simulink library "lib_LargeBuildingModel"  (R2026a)
settings: Solver=VariableStepAuto
libraries: WallSelector_lib x380, ExternalWall_lib x188, RoomWithAirVolume x140, fl_lib x139, RoomLevelControl_lib x1
(part 4 of 12)

== system lib_LargeBuildingModel/LargeBuildingModelLib/ConnectLevel3and4 ==
  note: Floor_A13R1(LivingRoom_A)
  note: Floor_A13R2(Bedroom_A)
  note: Floor_A13R3(Kitchen_A)
  note: Floor_A13R4(Bathroom_A)
  note: Floor_A13R5(FireExit_A)
  note: Floor_A13R6(Lobby1_A)
  note: Floor_A13R7(Lobby2_A)
  note: Floor_A14R1(LivingRoom_B)
  note: Floor_A14R2(Bedroom_B)
  note: Floor_A14R3(Kitchen_B)
  note: Floor_A14R4(Bathroom_B)
  note: Floor_A14R5(FireExit_B)
  note: Floor_A14R6(Lobby1_B)
  note: Floor_A14R7(Lobby2_B)
  note: Floor_A15R1(LivingRoom_C)
  note: Floor_A15R2(Bedroom_C)
  note: Floor_A15R3(Kitchen_C)
  note: Floor_A15R4(Bathroom_C)
  note: Floor_A15R5(FireExit_C)
  note: Floor_A15R6(Lobby1_C)
  note: Floor_A15R7(Lobby2_C)
  note: Floor_A16R1(LivingRoom_D)
  note: Floor_A16R2(Bedroom_D)
  note: Floor_A16R3(Kitchen_D)
  note: Floor_A16R4(Bathroom_D)
  note: Floor_A16R5(FireExit_D)
  note: Floor_A16R6(Lobby1_D)
  note: Floor_A16R7(Lobby2_D)
  ArrayBottom : SimscapeArrayConnection  Domain=foundation.thermal.thermal  ConcatenateDimension=1  NumScalarElements=28
  ArrayTop : SimscapeArrayConnection  Domain=foundation.thermal.thermal  ConcatenateDimension=1  NumScalarElements=28
  Floor_A13R1(LivingRoom_A)Blk : WallSelector_lib/Wall Selector  optWall=wallModelOption.wallOnly  wallLength=2.4384 % Parameterized on : 13-Jun-2026 10:47:16 m  wallHeight=4.572 % Parameterized on : 13-Jun-2026 10:47:16 m  wallThickness=0.03 % Parameterized on : 13-Jun-2026 10:47:16 m  wallMaterialDen=1400 % Parameterized on : 13-Jun-2026 10:47:30 kg/m^3  wallMaterialCp=1000 % Parameterized on : 13-Jun-2026 10:47:30 J/(K*kg)  wallAbsorptivity=0.5  wallThermalK=0.7 % Parameterized on : 13-Jun-2026 10:47:30 W/(K*m)  winLength=1 m  winHeight=0.5 m  winThickness=0.007 m  winMaterialDen=2500 kg/m^3  winMaterialCp=787 J/(K*kg)  winAbsorptivity=0.35  winThermalK=1 W/(K*m)  winTransmissivity=0.45  ventLength=0.1 m  ventHeight=0.1 m  extToWallHTC=30 % Parameterized on : 13-Jun-2026 10:47:30 W/(K*m^2)  intToRoomHTC=30 % Parameterized on : 13-Jun-2026 10:47:30 W/(K*m^2)  iniT=300 % Parameterized on : 13-Jun-2026 10:47:30 K
  Floor_A13R2(Bedroom_A)Blk : WallSelector_lib/Wall Selector  optWall=wallModelOption.wallOnly  wallLength=4.2672 % Parameterized on : 13-Jun-2026 10:47:16 m  wallHeight=4.572 % Parameterized on : 13-Jun-2026 10:47:16 m  wallThickness=0.03 % Parameterized on : 13-Jun-2026 10:47:16 m  wallMaterialDen=1400 % Parameterized on : 13-Jun-2026 10:47:30 kg/m^3  wallMaterialCp=1000 % Parameterized on : 13-Jun-2026 10:47:30 J/(K*kg)  wallAbsorptivity=0.5  wallThermalK=0.7 % Parameterized on : 13-Jun-2026 10:47:30 W/(K*m)  winLength=1 m  winHeight=0.5 m  winThickness=0.007 m  winMaterialDen=2500 kg/m^3  winMaterialCp=787 J/(K*kg)  winAbsorptivity=0.35  winThermalK=1 W/(K*m)  winTransmissivity=0.45  ventLength=0.1 m  ventHeight=0.1 m  extToWallHTC=30 % Parameterized on : 13-Jun-2026 10:47:30 W/(K*m^2)  intToRoomHTC=30 % Parameterized on : 13-Jun-2026 10:47:30 W/(K*m^2)  iniT=300 % Parameterized on : 13-Jun-2026 10:47:30 K
  Floor_A13R3(Kitchen_A)Blk : WallSelector_lib/Wall Selector  optWall=wallModelOption.wallOnly  wallLength=2.7432 % Parameterized on : 13-Jun-2026 10:47:16 m  wallHeight=3.9624 % Parameterized on : 13-Jun-2026 10:47:16 m  wallThickness=0.03 % Parameterized on : 13-Jun-2026 10:47:16 m  wallMaterialDen=1400 % Parameterized on : 13-Jun-2026 10:47:30 kg/m^3  wallMaterialCp=1000 % Parameterized on : 13-Jun-2026 10:47:30 J/(K*kg)  wallAbsorptivity=0.5  wallThermalK=0.7 % Parameterized on : 13-Jun-2026 10:47:30 W/(K*m)  winLength=1 m  winHeight=0.5 m  winThickness=0.007 m  winMaterialDen=2500 kg/m^3  winMaterialCp=787 J/(K*kg)  winAbsorptivity=0.35  winThermalK=1 W/(K*m)  winTransmissivity=0.45  ventLength=0.1 m  ventHeight=0.1 m  extToWallHTC=30 % Parameterized on : 13-Jun-2026 10:47:30 W/(K*m^2)  intToRoomHTC=30 % Parameterized on : 13-Jun-2026 10:47:30 W/(K*m^2)  iniT=300 % Parameterized on : 13-Jun-2026 10:47:30 K
  Floor_A13R4(Bathroom_A)Blk : WallSelector_lib/Wall Selector  optWall=wallModelOption.wallOnly  wallLength=2.4384 % Parameterized on : 13-Jun-2026 10:47:16 m  wallHeight=3.6576 % Parameterized on : 13-Jun-2026 10:47:16 m  wallThickness=0.03 % Parameterized on : 13-Jun-2026 10:47:16 m  wallMaterialDen=1400 % Parameterized on : 13-Jun-2026 10:47:30 kg/m^3  wallMaterialCp=1000 % Parameterized on : 13-Jun-2026 10:47:30 J/(K*kg)  wallAbsorptivity=0.5  wallThermalK=0.7 % Parameterized on : 13-Jun-2026 10:47:30 W/(K*m)  winLength=1 m  winHeight=0.5 m  winThickness=0.007 m  winMaterialDen=2500 kg/m^3  winMaterialCp=787 J/(K*kg)  winAbsorptivity=0.35  winThermalK=1 W/(K*m)  winTransmissivity=0.45  ventLength=0.1 m  ventHeight=0.1 m  extToWallHTC=30 % Parameterized on : 13-Jun-2026 10:47:30 W/(K*m^2)  intToRoomHTC=30 % Parameterized on : 13-Jun-2026 10:47:30 W/(K*m^2)  iniT=300 % Parameterized on : 13-Jun-2026 10:47:30 K
  Floor_A13R5(FireExit_A)Blk : WallSelector_lib/Wall Selector  optWall=wallModelOption.wallOnly  wallLength=1.8288 % Parameterized on : 13-Jun-2026 10:47:16 m  wallHeight=2.1336 % Parameterized on : 13-Jun-2026 10:47:16 m  wallThickness=0.03 % Parameterized on : 13-Jun-2026 10:47:16 m  wallMaterialDen=1400 % Parameterized on : 13-Jun-2026 10:47:30 kg/m^3  wallMaterialCp=1000 % Parameterized on : 13-Jun-2026 10:47:30 J/(K*kg)  wallAbsorptivity=0.5  wallThermalK=0.7 % Parameterized on : 13-Jun-2026 10:47:30 W/(K*m)  winLength=1 m  winHeight=0.5 m  winThickness=0.007 m  winMaterialDen=2500 kg/m^3  winMaterialCp=787 J/(K*kg)  winAbsorptivity=0.35  winThermalK=1 W/(K*m)  winTransmissivity=0.45  ventLength=0.1 m  ventHeight=0.1 m  extToWallHTC=30 % Parameterized on : 13-Jun-2026 10:47:30 W/(K*m^2)  intToRoomHTC=30 % Parameterized on : 13-Jun-2026 10:47:30 W/(K*m^2)  iniT=300 % Parameterized on : 13-Jun-2026 10:47:30 K
  Floor_A13R6(Lobby1_A)Blk : WallSelector_lib/Wall Selector  optWall=wallModelOption.wallOnly  wallLength=2.4384 % Parameterized on : 13-Jun-2026 10:47:16 m  wallHeight=2.4384 % Parameterized on : 13-Jun-2026 10:47:16 m  wallThickness=0.03 % Parameterized on : 13-Jun-2026 10:47:16 m  wallMaterialDen=1400 % Parameterized on : 13-Jun-2026 10:47:30 kg/m^3  wallMaterialCp=1000 % Parameterized on : 13-Jun-2026 10:47:30 J/(K*kg)  wallAbsorptivity=0.5  wallThermalK=0.7 % Parameterized on : 13-Jun-2026 10:47:30 W/(K*m)  winLength=1 m  winHeight=0.5 m  winThickness=0.007 m  winMaterialDen=2500 kg/m^3  winMaterialCp=787 J/(K*kg)  winAbsorptivity=0.35  winThermalK=1 W/(K*m)  winTransmissivity=0.45  ventLength=0.1 m  ventHeight=0.1 m  extToWallHTC=30 % Parameterized on : 13-Jun-2026 10:47:30 W/(K*m^2)  intToRoomHTC=30 % Parameterized on : 13-Jun-2026 10:47:30 W/(K*m^2)  iniT=300 % Parameterized on : 13-Jun-2026 10:47:30 K
  Floor_A13R7(Lobby2_A)Blk : WallSelector_lib/Wall Selector  optWall=wallModelOption.wallOnly  wallLength=2.4384 % Parameterized on : 13-Jun-2026 10:47:16 m  wallHeight=1.524 % Parameterized on : 13-Jun-2026 10:47:16 m  wallThickness=0.03 % Parameterized on : 13-Jun-2026 10:47:16 m  wallMaterialDen=1400 % Parameterized on : 13-Jun-2026 10:47:30 kg/m^3  wallMaterialCp=1000 % Parameterized on : 13-Jun-2026 10:47:30 J/(K*kg)  wallAbsorptivity=0.5  wallThermalK=0.7 % Parameterized on : 13-Jun-2026 10:47:30 W/(K*m)  winLength=1 m  winHeight=0.5 m  winThickness=0.007 m  winMaterialDen=2500 kg/m^3  winMaterialCp=787 J/(K*kg)  winAbsorptivity=0.35  winThermalK=1 W/(K*m)  winTransmissivity=0.45  ventLength=0.1 m  ventHeight=0.1 m  extToWallHTC=30 % Parameterized on : 13-Jun-2026 10:47:30 W/(K*m^2)  intToRoomHTC=30 % Parameterized on : 13-Jun-2026 10:47:30 W/(K*m^2)  iniT=300 % Parameterized on : 13-Jun-2026 10:47:30 K
  Floor_A14R1(LivingRoom_B)Blk : WallSelector_lib/Wall Selector  optWall=wallModelOption.wallOnly  wallLength=2.4384 % Parameterized on : 13-Jun-2026 10:47:16 m  wallHeight=4.572 % Parameterized on : 13-Jun-2026 10:47:16 m  wallThickness=0.03 % Parameterized on : 13-Jun-2026 10:47:16 m  wallMaterialDen=1400 % Parameterized on : 13-Jun-2026 10:47:30 kg/m^3  wallMaterialCp=1000 % Parameterized on : 13-Jun-2026 10:47:30 J/(K*kg)  wallAbsorptivity=0.5  wallThermalK=0.7 % Parameterized on : 13-Jun-2026 10:47:30 W/(K*m)  winLength=1 m  winHeight=0.5 m  winThickness=0.007 m  winMaterialDen=2500 kg/m^3  winMaterialCp=787 J/(K*kg)  winAbsorptivity=0.35  winThermalK=1 W/(K*m)  winTransmissivity=0.45  ventLength=0.1 m  ventHeight=0.1 m  extToWallHTC=30 % Parameterized on : 13-Jun-2026 10:47:30 W/(K*m^2)  intToRoomHTC=30 % Parameterized on : 13-Jun-2026 10:47:30 W/(K*m^2)  iniT=300 % Parameterized on : 13-Jun-2026 10:47:30 K
  Floor_A14R2(Bedroom_B)Blk : WallSelector_lib/Wall Selector  optWall=wallModelOption.wallOnly  wallLength=4.2672 % Parameterized on : 13-Jun-2026 10:47:16 m  wallHeight=4.572 % Parameterized on : 13-Jun-2026 10:47:16 m  wallThickness=0.03 % Parameterized on : 13-Jun-2026 10:47:16 m  wallMaterialDen=1400 % Parameterized on : 13-Jun-2026 10:47:30 kg/m^3  wallMaterialCp=1000 % Parameterized on : 13-Jun-2026 10:47:30 J/(K*kg)  wallAbsorptivity=0.5  wallThermalK=0.7 % Parameterized on : 13-Jun-2026 10:47:30 W/(K*m)  winLength=1 m  winHeight=0.5 m  winThickness=0.007 m  winMaterialDen=2500 kg/m^3  winMaterialCp=787 J/(K*kg)  winAbsorptivity=0.35  winThermalK=1 W/(K*m)  winTransmissivity=0.45  ventLength=0.1 m  ventHeight=0.1 m  extToWallHTC=30 % Parameterized on : 13-Jun-2026 10:47:30 W/(K*m^2)  intToRoomHTC=30 % Parameterized on : 13-Jun-2026 10:47:30 W/(K*m^2)  iniT=300 % Parameterized on : 13-Jun-2026 10:47:30 K
  Floor_A14R3(Kitchen_B)Blk : WallSelector_lib/Wall Selector  optWall=wallModelOption.wallOnly  wallLength=2.7432 % Parameterized on : 13-Jun-2026 10:47:16 m  wallHeight=3.9624 % Parameterized on : 13-Jun-2026 10:47:16 m  wallThickness=0.03 % Parameterized on : 13-Jun-2026 10:47:16 m  wallMaterialDen=1400 % Parameterized on : 13-Jun-2026 10:47:30 kg/m^3  wallMaterialCp=1000 % Parameterized on : 13-Jun-2026 10:47:30 J/(K*kg)  wallAbsorptivity=0.5  wallThermalK=0.7 % Parameterized on : 13-Jun-2026 10:47:30 W/(K*m)  winLength=1 m  winHeight=0.5 m  winThickness=0.007 m  winMaterialDen=2500 kg/m^3  winMaterialCp=787 J/(K*kg)  winAbsorptivity=0.35  winThermalK=1 W/(K*m)  winTransmissivity=0.45  ventLength=0.1 m  ventHeight=0.1 m  extToWallHTC=30 % Parameterized on : 13-Jun-2026 10:47:30 W/(K*m^2)  intToRoomHTC=30 % Parameterized on : 13-Jun-2026 10:47:30 W/(K*m^2)  iniT=300 % Parameterized on : 13-Jun-2026 10:47:30 K
  Floor_A14R4(Bathroom_B)Blk : WallSelector_lib/Wall Selector  optWall=wallModelOption.wallOnly  wallLength=2.4384 % Parameterized on : 13-Jun-2026 10:47:16 m  wallHeight=3.6576 % Parameterized on : 13-Jun-2026 10:47:16 m  wallThickness=0.03 % Parameterized on : 13-Jun-2026 10:47:16 m  wallMaterialDen=1400 % Parameterized on : 13-Jun-2026 10:47:30 kg/m^3  wallMaterialCp=1000 % Parameterized on : 13-Jun-2026 10:47:30 J/(K*kg)  wallAbsorptivity=0.5  wallThermalK=0.7 % Parameterized on : 13-Jun-2026 10:47:30 W/(K*m)  winLength=1 m  winHeight=0.5 m  winThickness=0.007 m  winMaterialDen=2500 kg/m^3  winMaterialCp=787 J/(K*kg)  winAbsorptivity=0.35  winThermalK=1 W/(K*m)  winTransmissivity=0.45  ventLength=0.1 m  ventHeight=0.1 m  extToWallHTC=30 % Parameterized on : 13-Jun-2026 10:47:30 W/(K*m^2)  intToRoomHTC=30 % Parameterized on : 13-Jun-2026 10:47:30 W/(K*m^2)  iniT=300 % Parameterized on : 13-Jun-2026 10:47:30 K
  Floor_A14R5(FireExit_B)Blk : WallSelector_lib/Wall Selector  optWall=wallModelOption.wallOnly  wallLength=1.8288 % Parameterized on : 13-Jun-2026 10:47:16 m  wallHeight=2.1336 % Parameterized on : 13-Jun-2026 10:47:16 m  wallThickness=0.03 % Parameterized on : 13-Jun-2026 10:47:16 m  wallMaterialDen=1400 % Parameterized on : 13-Jun-2026 10:47:30 kg/m^3  wallMaterialCp=1000 % Parameterized on : 13-Jun-2026 10:47:30 J/(K*kg)  wallAbsorptivity=0.5  wallThermalK=0.7 % Parameterized on : 13-Jun-2026 10:47:30 W/(K*m)  winLength=1 m  winHeight=0.5 m  winThickness=0.007 m  winMaterialDen=2500 kg/m^3  winMaterialCp=787 J/(K*kg)  winAbsorptivity=0.35  winThermalK=1 W/(K*m)  winTransmissivity=0.45  ventLength=0.1 m  ventHeight=0.1 m  extToWallHTC=30 % Parameterized on : 13-Jun-2026 10:47:30 W/(K*m^2)  intToRoomHTC=30 % Parameterized on : 13-Jun-2026 10:47:30 W/(K*m^2)  iniT=300 % Parameterized on : 13-Jun-2026 10:47:30 K
  Floor_A14R6(Lobby1_B)Blk : WallSelector_lib/Wall Selector  optWall=wallModelOption.wallOnly  wallLength=2.4384 % Parameterized on : 13-Jun-2026 10:47:16 m  wallHeight=2.4384 % Parameterized on : 13-Jun-2026 10:47:16 m  wallThickness=0.03 % Parameterized on : 13-Jun-2026 10:47:16 m  wallMaterialDen=1400 % Parameterized on : 13-Jun-2026 10:47:30 kg/m^3  wallMaterialCp=1000 % Parameterized on : 13-Jun-2026 10:47:30 J/(K*kg)  wallAbsorptivity=0.5  wallThermalK=0.7 % Parameterized on : 13-Jun-2026 10:47:30 W/(K*m)  winLength=1 m  winHeight=0.5 m  winThickness=0.007 m  winMaterialDen=2500 kg/m^3  winMaterialCp=787 J/(K*kg)  winAbsorptivity=0.35  winThermalK=1 W/(K*m)  winTransmissivity=0.45  ventLength=0.1 m  ventHeight=0.1 m  extToWallHTC=30 % Parameterized on : 13-Jun-2026 10:47:30 W/(K*m^2)  intToRoomHTC=30 % Parameterized on : 13-Jun-2026 10:47:30 W/(K*m^2)  iniT=300 % Parameterized on : 13-Jun-2026 10:47:30 K
  Floor_A14R7(Lobby2_B)Blk : WallSelector_lib/Wall Selector  optWall=wallModelOption.wallOnly  wallLength=2.4384 % Parameterized on : 13-Jun-2026 10:47:16 m  wallHeight=1.524 % Parameterized on : 13-Jun-2026 10:47:16 m  wallThickness=0.03 % Parameterized on : 13-Jun-2026 10:47:16 m  wallMaterialDen=1400 % Parameterized on : 13-Jun-2026 10:47:30 kg/m^3  wallMaterialCp=1000 % Parameterized on : 13-Jun-2026 10:47:30 J/(K*kg)  wallAbsorptivity=0.5  wallThermalK=0.7 % Parameterized on : 13-Jun-2026 10:47:30 W/(K*m)  winLength=1 m  winHeight=0.5 m  winThickness=0.007 m  winMaterialDen=2500 kg/m^3  winMaterialCp=787 J/(K*kg)  winAbsorptivity=0.35  winThermalK=1 W/(K*m)  winTransmissivity=0.45  ventLength=0.1 m  ventHeight=0.1 m  extToWallHTC=30 % Parameterized on : 13-Jun-2026 10:47:30 W/(K*m^2)  intToRoomHTC=30 % Parameterized on : 13-Jun-2026 10:47:30 W/(K*m^2)  iniT=300 % Parameterized on : 13-Jun-2026 10:47:30 K
  Floor_A15R1(LivingRoom_C)Blk : WallSelector_lib/Wall Selector  optWall=wallModelOption.wallOnly  wallLength=2.4384 % Parameterized on : 13-Jun-2026 10:47:16 m  wallHeight=4.572 % Parameterized on : 13-Jun-2026 10:47:16 m  wallThickness=0.03 % Parameterized on : 13-Jun-2026 10:47:16 m  wallMaterialDen=1400 % Parameterized on : 13-Jun-2026 10:47:30 kg/m^3  wallMaterialCp=1000 % Parameterized on : 13-Jun-2026 10:47:30 J/(K*kg)  wallAbsorptivity=0.5  wallThermalK=0.7 % Parameterized on : 13-Jun-2026 10:47:30 W/(K*m)  winLength=1 m  winHeight=0.5 m  winThickness=0.007 m  winMaterialDen=2500 kg/m^3  winMaterialCp=787 J/(K*kg)  winAbsorptivity=0.35  winThermalK=1 W/(K*m)  winTransmissivity=0.45  ventLength=0.1 m  ventHeight=0.1 m  extToWallHTC=30 % Parameterized on : 13-Jun-2026 10:47:30 W/(K*m^2)  intToRoomHTC=30 % Parameterized on : 13-Jun-2026 10:47:30 W/(K*m^2)  iniT=300 % Parameterized on : 13-Jun-2026 10:47:30 K
  Floor_A15R2(Bedroom_C)Blk : WallSelector_lib/Wall Selector  optWall=wallModelOption.wallOnly  wallLength=4.2672 % Parameterized on : 13-Jun-2026 10:47:16 m  wallHeight=4.572 % Parameterized on : 13-Jun-2026 10:47:16 m  wallThickness=0.03 % Parameterized on : 13-Jun-2026 10:47:16 m  wallMaterialDen=1400 % Parameterized on : 13-Jun-2026 10:47:30 kg/m^3  wallMaterialCp=1000 % Parameterized on : 13-Jun-2026 10:47:30 J/(K*kg)  wallAbsorptivity=0.5  wallThermalK=0.7 % Parameterized on : 13-Jun-2026 10:47:30 W/(K*m)  winLength=1 m  winHeight=0.5 m  winThickness=0.007 m  winMaterialDen=2500 kg/m^3  winMaterialCp=787 J/(K*kg)  winAbsorptivity=0.35  winThermalK=1 W/(K*m)  winTransmissivity=0.45  ventLength=0.1 m  ventHeight=0.1 m  extToWallHTC=30 % Parameterized on : 13-Jun-2026 10:47:30 W/(K*m^2)  intToRoomHTC=30 % Parameterized on : 13-Jun-2026 10:47:30 W/(K*m^2)  iniT=300 % Parameterized on : 13-Jun-2026 10:47:30 K
  Floor_A15R3(Kitchen_C)Blk : WallSelector_lib/Wall Selector  optWall=wallModelOption.wallOnly  wallLength=2.7432 % Parameterized on : 13-Jun-2026 10:47:16 m  wallHeight=3.9624 % Parameterized on : 13-Jun-2026 10:47:16 m  wallThickness=0.03 % Parameterized on : 13-Jun-2026 10:47:16 m  wallMaterialDen=1400 % Parameterized on : 13-Jun-2026 10:47:30 kg/m^3  wallMaterialCp=1000 % Parameterized on : 13-Jun-2026 10:47:30 J/(K*kg)  wallAbsorptivity=0.5  wallThermalK=0.7 % Parameterized on : 13-Jun-2026 10:47:30 W/(K*m)  winLength=1 m  winHeight=0.5 m  winThickness=0.007 m  winMaterialDen=2500 kg/m^3  winMaterialCp=787 J/(K*kg)  winAbsorptivity=0.35  winThermalK=1 W/(K*m)  winTransmissivity=0.45  ventLength=0.1 m  ventHeight=0.1 m  extToWallHTC=30 % Parameterized on : 13-Jun-2026 10:47:30 W/(K*m^2)  intToRoomHTC=30 % Parameterized on : 13-Jun-2026 10:47:30 W/(K*m^2)  iniT=300 % Parameterized on : 13-Jun-2026 10:47:30 K
  Floor_A15R4(Bathroom_C)Blk : WallSelector_lib/Wall Selector  optWall=wallModelOption.wallOnly  wallLength=2.4384 % Parameterized on : 13-Jun-2026 10:47:16 m  wallHeight=3.6576 % Parameterized on : 13-Jun-2026 10:47:16 m  wallThickness=0.03 % Parameterized on : 13-Jun-2026 10:47:16 m  wallMaterialDen=1400 % Parameterized on : 13-Jun-2026 10:47:30 kg/m^3  wallMaterialCp=1000 % Parameterized on : 13-Jun-2026 10:47:30 J/(K*kg)  wallAbsorptivity=0.5  wallThermalK=0.7 % Parameterized on : 13-Jun-2026 10:47:30 W/(K*m)  winLength=1 m  winHeight=0.5 m  winThickness=0.007 m  winMaterialDen=2500 kg/m^3  winMaterialCp=787 J/(K*kg)  winAbsorptivity=0.35  winThermalK=1 W/(K*m)  winTransmissivity=0.45  ventLength=0.1 m  ventHeight=0.1 m  extToWallHTC=30 % Parameterized on : 13-Jun-2026 10:47:30 W/(K*m^2)  intToRoomHTC=30 % Parameterized on : 13-Jun-2026 10:47:30 W/(K*m^2)  iniT=300 % Parameterized on : 13-Jun-2026 10:47:30 K
  Floor_A15R5(FireExit_C)Blk : WallSelector_lib/Wall Selector  optWall=wallModelOption.wallOnly  wallLength=1.8288 % Parameterized on : 13-Jun-2026 10:47:16 m  wallHeight=2.1336 % Parameterized on : 13-Jun-2026 10:47:16 m  wallThickness=0.03 % Parameterized on : 13-Jun-2026 10:47:16 m  wallMaterialDen=1400 % Parameterized on : 13-Jun-2026 10:47:30 kg/m^3  wallMaterialCp=1000 % Parameterized on : 13-Jun-2026 10:47:30 J/(K*kg)  wallAbsorptivity=0.5  wallThermalK=0.7 % Parameterized on : 13-Jun-2026 10:47:30 W/(K*m)  winLength=1 m  winHeight=0.5 m  winThickness=0.007 m  winMaterialDen=2500 kg/m^3  winMaterialCp=787 J/(K*kg)  winAbsorptivity=0.35  winThermalK=1 W/(K*m)  winTransmissivity=0.45  ventLength=0.1 m  ventHeight=0.1 m  extToWallHTC=30 % Parameterized on : 13-Jun-2026 10:47:30 W/(K*m^2)  intToRoomHTC=30 % Parameterized on : 13-Jun-2026 10:47:30 W/(K*m^2)  iniT=300 % Parameterized on : 13-Jun-2026 10:47:30 K
  Floor_A15R6(Lobby1_C)Blk : WallSelector_lib/Wall Selector  optWall=wallModelOption.wallOnly  wallLength=2.4384 % Parameterized on : 13-Jun-2026 10:47:16 m  wallHeight=2.4384 % Parameterized on : 13-Jun-2026 10:47:16 m  wallThickness=0.03 % Parameterized on : 13-Jun-2026 10:47:16 m  wallMaterialDen=1400 % Parameterized on : 13-Jun-2026 10:47:30 kg/m^3  wallMaterialCp=1000 % Parameterized on : 13-Jun-2026 10:47:30 J/(K*kg)  wallAbsorptivity=0.5  wallThermalK=0.7 % Parameterized on : 13-Jun-2026 10:47:30 W/(K*m)  winLength=1 m  winHeight=0.5 m  winThickness=0.007 m  winMaterialDen=2500 kg/m^3  winMaterialCp=787 J/(K*kg)  winAbsorptivity=0.35  winThermalK=1 W/(K*m)  winTransmissivity=0.45  ventLength=0.1 m  ventHeight=0.1 m  extToWallHTC=30 % Parameterized on : 13-Jun-2026 10:47:30 W/(K*m^2)  intToRoomHTC=30 % Parameterized on : 13-Jun-2026 10:47:30 W/(K*m^2)  iniT=300 % Parameterized on : 13-Jun-2026 10:47:30 K
  Floor_A15R7(Lobby2_C)Blk : WallSelector_lib/Wall Selector  optWall=wallModelOption.wallOnly  wallLength=2.4384 % Parameterized on : 13-Jun-2026 10:47:16 m  wallHeight=1.524 % Parameterized on : 13-Jun-2026 10:47:16 m  wallThickness=0.03 % Parameterized on : 13-Jun-2026 10:47:16 m  wallMaterialDen=1400 % Parameterized on : 13-Jun-2026 10:47:30 kg/m^3  wallMaterialCp=1000 % Parameterized on : 13-Jun-2026 10:47:30 J/(K*kg)  wallAbsorptivity=0.5  wallThermalK=0.7 % Parameterized on : 13-Jun-2026 10:47:30 W/(K*m)  winLength=1 m  winHeight=0.5 m  winThickness=0.007 m  winMaterialDen=2500 kg/m^3  winMaterialCp=787 J/(K*kg)  winAbsorptivity=0.35  winThermalK=1 W/(K*m)  winTransmissivity=0.45  ventLength=0.1 m  ventHeight=0.1 m  extToWallHTC=30 % Parameterized on : 13-Jun-2026 10:47:30 W/(K*m^2)  intToRoomHTC=30 % Parameterized on : 13-Jun-2026 10:47:30 W/(K*m^2)  iniT=300 % Parameterized on : 13-Jun-2026 10:47:30 K
  Floor_A16R1(LivingRoom_D)Blk : WallSelector_lib/Wall Selector  optWall=wallModelOption.wallOnly  wallLength=2.4384 % Parameterized on : 13-Jun-2026 10:47:16 m  wallHeight=4.572 % Parameterized on : 13-Jun-2026 10:47:16 m  wallThickness=0.03 % Parameterized on : 13-Jun-2026 10:47:16 m  wallMaterialDen=1400 % Parameterized on : 13-Jun-2026 10:47:30 kg/m^3  wallMaterialCp=1000 % Parameterized on : 13-Jun-2026 10:47:30 J/(K*kg)  wallAbsorptivity=0.5  wallThermalK=0.7 % Parameterized on : 13-Jun-2026 10:47:30 W/(K*m)  winLength=1 m  winHeight=0.5 m  winThickness=0.007 m  winMaterialDen=2500 kg/m^3  winMaterialCp=787 J/(K*kg)  winAbsorptivity=0.35  winThermalK=1 W/(K*m)  winTransmissivity=0.45  ventLength=0.1 m  ventHeight=0.1 m  extToWallHTC=30 % Parameterized on : 13-Jun-2026 10:47:30 W/(K*m^2)  intToRoomHTC=30 % Parameterized on : 13-Jun-2026 10:47:30 W/(K*m^2)  iniT=300 % Parameterized on : 13-Jun-2026 10:47:30 K
  Floor_A16R2(Bedroom_D)Blk : WallSelector_lib/Wall Selector  optWall=wallModelOption.wallOnly  wallLength=4.2672 % Parameterized on : 13-Jun-2026 10:47:16 m  wallHeight=4.572 % Parameterized on : 13-Jun-2026 10:47:16 m  wallThickness=0.03 % Parameterized on : 13-Jun-2026 10:47:16 m  wallMaterialDen=1400 % Parameterized on : 13-Jun-2026 10:47:30 kg/m^3  wallMaterialCp=1000 % Parameterized on : 13-Jun-2026 10:47:30 J/(K*kg)  wallAbsorptivity=0.5  wallThermalK=0.7 % Parameterized on : 13-Jun-2026 10:47:30 W/(K*m)  winLength=1 m  winHeight=0.5 m  winThickness=0.007 m  winMaterialDen=2500 kg/m^3  winMaterialCp=787 J/(K*kg)  winAbsorptivity=0.35  winThermalK=1 W/(K*m)  winTransmissivity=0.45  ventLength=0.1 m  ventHeight=0.1 m  extToWallHTC=30 % Parameterized on : 13-Jun-2026 10:47:30 W/(K*m^2)  intToRoomHTC=30 % Parameterized on : 13-Jun-2026 10:47:30 W/(K*m^2)  iniT=300 % Parameterized on : 13-Jun-2026 10:47:30 K
  Floor_A16R3(Kitchen_D)Blk : WallSelector_lib/Wall Selector  optWall=wallModelOption.wallOnly  wallLength=2.7432 % Parameterized on : 13-Jun-2026 10:47:16 m  wallHeight=3.9624 % Parameterized on : 13-Jun-2026 10:47:16 m  wallThickness=0.03 % Parameterized on : 13-Jun-2026 10:47:16 m  wallMaterialDen=1400 % Parameterized on : 13-Jun-2026 10:47:30 kg/m^3  wallMaterialCp=1000 % Parameterized on : 13-Jun-2026 10:47:30 J/(K*kg)  wallAbsorptivity=0.5  wallThermalK=0.7 % Parameterized on : 13-Jun-2026 10:47:30 W/(K*m)  winLength=1 m  winHeight=0.5 m  winThickness=0.007 m  winMaterialDen=2500 kg/m^3  winMaterialCp=787 J/(K*kg)  winAbsorptivity=0.35  winThermalK=1 W/(K*m)  winTransmissivity=0.45  ventLength=0.1 m  ventHeight=0.1 m  extToWallHTC=30 % Parameterized on : 13-Jun-2026 10:47:30 W/(K*m^2)  intToRoomHTC=30 % Parameterized on : 13-Jun-2026 10:47:30 W/(K*m^2)  iniT=300 % Parameterized on : 13-Jun-2026 10:47:30 K
  Floor_A16R4(Bathroom_D)Blk : WallSelector_lib/Wall Selector  optWall=wallModelOption.wallOnly  wallLength=2.4384 % Parameterized on : 13-Jun-2026 10:47:16 m  wallHeight=3.6576 % Parameterized on : 13-Jun-2026 10:47:16 m  wallThickness=0.03 % Parameterized on : 13-Jun-2026 10:47:16 m  wallMaterialDen=1400 % Parameterized on : 13-Jun-2026 10:47:30 kg/m^3  wallMaterialCp=1000 % Parameterized on : 13-Jun-2026 10:47:30 J/(K*kg)  wallAbsorptivity=0.5  wallThermalK=0.7 % Parameterized on : 13-Jun-2026 10:47:30 W/(K*m)  winLength=1 m  winHeight=0.5 m  winThickness=0.007 m  winMaterialDen=2500 kg/m^3  winMaterialCp=787 J/(K*kg)  winAbsorptivity=0.35  winThermalK=1 W/(K*m)  winTransmissivity=0.45  ventLength=0.1 m  ventHeight=0.1 m  extToWallHTC=30 % Parameterized on : 13-Jun-2026 10:47:30 W/(K*m^2)  intToRoomHTC=30 % Parameterized on : 13-Jun-2026 10:47:30 W/(K*m^2)  iniT=300 % Parameterized on : 13-Jun-2026 10:47:30 K
  Floor_A16R5(FireExit_D)Blk : WallSelector_lib/Wall Selector  optWall=wallModelOption.wallOnly  wallLength=1.8288 % Parameterized on : 13-Jun-2026 10:47:16 m  wallHeight=2.1336 % Parameterized on : 13-Jun-2026 10:47:16 m  wallThickness=0.03 % Parameterized on : 13-Jun-2026 10:47:16 m  wallMaterialDen=1400 % Parameterized on : 13-Jun-2026 10:47:30 kg/m^3  wallMaterialCp=1000 % Parameterized on : 13-Jun-2026 10:47:30 J/(K*kg)  wallAbsorptivity=0.5  wallThermalK=0.7 % Parameterized on : 13-Jun-2026 10:47:30 W/(K*m)  winLength=1 m  winHeight=0.5 m  winThickness=0.007 m  winMaterialDen=2500 kg/m^3  winMaterialCp=787 J/(K*kg)  winAbsorptivity=0.35  winThermalK=1 W/(K*m)  winTransmissivity=0.45  ventLength=0.1 m  ventHeight=0.1 m  extToWallHTC=30 % Parameterized on : 13-Jun-2026 10:47:30 W/(K*m^2)  intToRoomHTC=30 % Parameterized on : 13-Jun-2026 10:47:30 W/(K*m^2)  iniT=300 % Parameterized on : 13-Jun-2026 10:47:30 K
  Floor_A16R6(Lobby1_D)Blk : WallSelector_lib/Wall Selector  optWall=wallModelOption.wallOnly  wallLength=2.4384 % Parameterized on : 13-Jun-2026 10:47:16 m  wallHeight=2.4384 % Parameterized on : 13-Jun-2026 10:47:16 m  wallThickness=0.03 % Parameterized on : 13-Jun-2026 10:47:16 m  wallMaterialDen=1400 % Parameterized on : 13-Jun-2026 10:47:30 kg/m^3  wallMaterialCp=1000 % Parameterized on : 13-Jun-2026 10:47:30 J/(K*kg)  wallAbsorptivity=0.5  wallThermalK=0.7 % Parameterized on : 13-Jun-2026 10:47:30 W/(K*m)  winLength=1 m  winHeight=0.5 m  winThickness=0.007 m  winMaterialDen=2500 kg/m^3  winMaterialCp=787 J/(K*kg)  winAbsorptivity=0.35  winThermalK=1 W/(K*m)  winTransmissivity=0.45  ventLength=0.1 m  ventHeight=0.1 m  extToWallHTC=30 % Parameterized on : 13-Jun-2026 10:47:30 W/(K*m^2)  intToRoomHTC=30 % Parameterized on : 13-Jun-2026 10:47:30 W/(K*m^2)  iniT=300 % Parameterized on : 13-Jun-2026 10:47:30 K
  Floor_A16R7(Lobby2_D)Blk : WallSelector_lib/Wall Selector  optWall=wallModelOption.wallOnly  wallLength=2.4384 % Parameterized on : 13-Jun-2026 10:47:16 m  wallHeight=1.524 % Parameterized on : 13-Jun-2026 10:47:16 m  wallThickness=0.03 % Parameterized on : 13-Jun-2026 10:47:16 m  wallMaterialDen=1400 % Parameterized on : 13-Jun-2026 10:47:30 kg/m^3  wallMaterialCp=1000 % Parameterized on : 13-Jun-2026 10:47:30 J/(K*kg)  wallAbsorptivity=0.5  wallThermalK=0.7 % Parameterized on : 13-Jun-2026 10:47:30 W/(K*m)  winLength=1 m  winHeight=0.5 m  winThickness=0.007 m  winMaterialDen=2500 kg/m^3  winMaterialCp=787 J/(K*kg)  winAbsorptivity=0.35  winThermalK=1 W/(K*m)  winTransmissivity=0.45  ventLength=0.1 m  ventHeight=0.1 m  extToWallHTC=30 % Parameterized on : 13-Jun-2026 10:47:30 W/(K*m^2)  intToRoomHTC=30 % Parameterized on : 13-Jun-2026 10:47:30 W/(K*m^2)  iniT=300 % Parameterized on : 13-Jun-2026 10:47:30 K
  Top : PMIOPort  Side=Left
  Bottom : PMIOPort  Port=2  Side=Right
  connections:
  ArrayTop/RConn1 -- Top/RConn1
  Floor_A13R1(LivingRoom_A)Blk/LConn1 -- ArrayTop/LConn1
  Floor_A13R2(Bedroom_A)Blk/LConn1 -- ArrayTop/LConn2
  Floor_A13R3(Kitchen_A)Blk/LConn1 -- ArrayTop/LConn3
  Floor_A13R4(Bathroom_A)Blk/LConn1 -- ArrayTop/LConn4
  Floor_A13R5(FireExit_A)Blk/LConn1 -- ArrayTop/LConn5
  Floor_A13R6(Lobby1_A)Blk/LConn1 -- ArrayTop/LConn6
  Floor_A13R7(Lobby2_A)Blk/LConn1 -- ArrayTop/LConn7
  Floor_A14R1(LivingRoom_B)Blk/LConn1 -- ArrayTop/LConn8
  Floor_A14R2(Bedroom_B)Blk/LConn1 -- ArrayTop/LConn9
  Floor_A14R3(Kitchen_B)Blk/LConn1 -- ArrayTop/LConn10
  Floor_A14R4(Bathroom_B)Blk/LConn1 -- ArrayTop/LConn11
  Floor_A14R5(FireExit_B)Blk/LConn1 -- ArrayTop/LConn12
  Floor_A14R6(Lobby1_B)Blk/LConn1 -- ArrayTop/LConn13
  Floor_A14R7(Lobby2_B)Blk/LConn1 -- ArrayTop/LConn14
  Floor_A15R1(LivingRoom_C)Blk/LConn1 -- ArrayTop/LConn15
  Floor_A15R2(Bedroom_C)Blk/LConn1 -- ArrayTop/LConn16
  Floor_A15R3(Kitchen_C)Blk/LConn1 -- ArrayTop/LConn17
  Floor_A15R4(Bathroom_C)Blk/LConn1 -- ArrayTop/LConn18
  Floor_A15R5(FireExit_C)Blk/LConn1 -- ArrayTop/LConn19
  Floor_A15R6(Lobby1_C)Blk/LConn1 -- ArrayTop/LConn20
  Floor_A15R7(Lobby2_C)Blk/LConn1 -- ArrayTop/LConn21
  Floor_A16R1(LivingRoom_D)Blk/LConn1 -- ArrayTop/LConn22
  Floor_A16R2(Bedroom_D)Blk/LConn1 -- ArrayTop/LConn23
  Floor_A16R3(Kitchen_D)Blk/LConn1 -- ArrayTop/LConn24
  Floor_A16R4(Bathroom_D)Blk/LConn1 -- ArrayTop/LConn25
  Floor_A16R5(FireExit_D)Blk/LConn1 -- ArrayTop/LConn26
  Floor_A16R6(Lobby1_D)Blk/LConn1 -- ArrayTop/LConn27
  Floor_A16R7(Lobby2_D)Blk/LConn1 -- ArrayTop/LConn28
  ArrayBottom/RConn1 -- Bottom/RConn1
  Floor_A13R1(LivingRoom_A)Blk/RConn1 -- ArrayBottom/LConn1
  Floor_A13R2(Bedroom_A)Blk/RConn1 -- ArrayBottom/LConn2
  Floor_A13R3(Kitchen_A)Blk/RConn1 -- ArrayBottom/LConn3
  Floor_A13R4(Bathroom_A)Blk/RConn1 -- ArrayBottom/LConn4
  Floor_A13R5(FireExit_A)Blk/RConn1 -- ArrayBottom/LConn5
  Floor_A13R6(Lobby1_A)Blk/RConn1 -- ArrayBottom/LConn6
  Floor_A13R7(Lobby2_A)Blk/RConn1 -- ArrayBottom/LConn7
  Floor_A14R1(LivingRoom_B)Blk/RConn1 -- ArrayBottom/LConn8
  Floor_A14R2(Bedroom_B)Blk/RConn1 -- ArrayBottom/LConn9
  Floor_A14R3(Kitchen_B)Blk/RConn1 -- ArrayBottom/LConn10
  Floor_A14R4(Bathroom_B)Blk/RConn1 -- ArrayBottom/LConn11
  Floor_A14R5(FireExit_B)Blk/RConn1 -- ArrayBottom/LConn12
  Floor_A14R6(Lobby1_B)Blk/RConn1 -- ArrayBottom/LConn13
  Floor_A14R7(Lobby2_B)Blk/RConn1 -- ArrayBottom/LConn14
  Floor_A15R1(LivingRoom_C)Blk/RConn1 -- ArrayBottom/LConn15
  Floor_A15R2(Bedroom_C)Blk/RConn1 -- ArrayBottom/LConn16
  Floor_A15R3(Kitchen_C)Blk/RConn1 -- ArrayBottom/LConn17
  Floor_A15R4(Bathroom_C)Blk/RConn1 -- ArrayBottom/LConn18
  Floor_A15R5(FireExit_C)Blk/RConn1 -- ArrayBottom/LConn19
  Floor_A15R6(Lobby1_C)Blk/RConn1 -- ArrayBottom/LConn20
  Floor_A15R7(Lobby2_C)Blk/RConn1 -- ArrayBottom/LConn21
  Floor_A16R1(LivingRoom_D)Blk/RConn1 -- ArrayBottom/LConn22
  Floor_A16R2(Bedroom_D)Blk/RConn1 -- ArrayBottom/LConn23
  Floor_A16R3(Kitchen_D)Blk/RConn1 -- ArrayBottom/LConn24
  Floor_A16R4(Bathroom_D)Blk/RConn1 -- ArrayBottom/LConn25
  Floor_A16R5(FireExit_D)Blk/RConn1 -- ArrayBottom/LConn26
  Floor_A16R6(Lobby1_D)Blk/RConn1 -- ArrayBottom/LConn27
  Floor_A16R7(Lobby2_D)Blk/RConn1 -- ArrayBottom/LConn28
